simulink model "TCR_Model"  (R2026a)
settings: Solver=ode23t  StopTime=0.1  MaxStep=1e-5  RelTol=1e-4
model workspace (MAT data in the model file):
  Lr = 0.1
  PW = 60
  Rr = 0.1
  Vg = 10
  Vrms = 230
  alpha = 120
  f = 50
libraries: nesl_utility x7, fl_lib x6, ee_lib x4

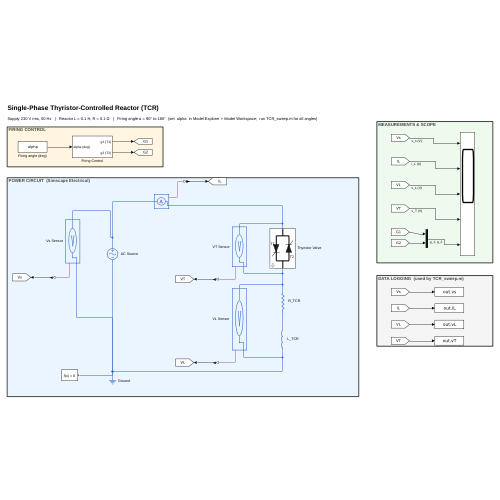
[thumbnail: Simulink's stored preview of the top-level diagram]
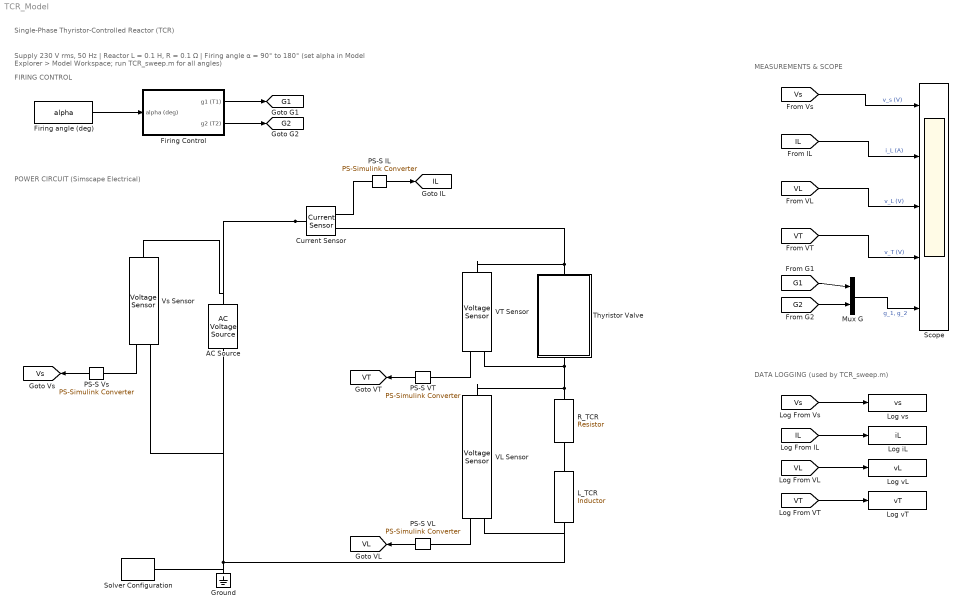
== system TCR_Model ==
  note: Single-Phase Thyristor-Controlled Reactor (TCR)
  note: Supply 230 V rms, 50 Hz | Reactor L = 0.1 H, R = 0.1 Ω | Firing angle α = 90° to 180° (set alpha in Model Explorer > Model Workspace; run TCR_sweep.m for all angles)
  note: FIRING CONTROL
  note: POWER CIRCUIT (Simscape Electrical)
  note: MEASUREMENTS & SCOPE
  note: DATA LOGGING (used by TCR_sweep.m)
  AC Source : fl_lib/Electrical/Electrical Sources/AC Voltage Source  amp=Vrms*sqrt(2) V  shift=0 deg  frequency=f Hz
  Current Sensor : fl_lib/Electrical/Electrical Sensors/Current Sensor
  Firing Control : Subsystem
  Firing angle (deg) : Constant  Value=alpha
  Ground : fl_lib/Electrical/Electrical Elements/Electrical Reference
  L_TCR : ee_lib/Passive/Inductor  l=Lr H  enable_L_tol=ee.enum.toleranceApplication.none  L_tol=20  tol_distribution=ee.enum.toleranceDistribution.uniform  nSigma=4  r=0 Ohm  g=1e-9 1/Ohm  enable_operating_limits=ee.enum.enable.no  operating_limit_action=ee.enum.passive.reportOpLim.warn  max_working_current=1 A  power_rating=1 W  i_L_specify=off  i_L_priority=High  i_L=0 A  i_L_nominal_specify=off  i_L_nominal_value=1  i_L_nominal_unit=A
  Log iL : ToWorkspace  VariableName=iL  SaveFormat=Timeseries  SampleTime=-1
  Log vL : ToWorkspace  VariableName=vL  SaveFormat=Timeseries  SampleTime=-1
  Log vT : ToWorkspace  VariableName=vT  SaveFormat=Timeseries  SampleTime=-1
  Log vs : ToWorkspace  VariableName=vs  SaveFormat=Timeseries  SampleTime=-1
  Mux G : Mux  Inputs=2
  PS-S IL : nesl_utility/PS-Simulink Converter  PhysicalDomain=network_engine_domain  SubClassName=ps_output  LeftPortType=input  RightPortType=output  PseudoPeriodic=off  Frequencies=[]  VectorFormat=inherit  Unit=inherit  AffineConversion=off
  PS-S VL : nesl_utility/PS-Simulink Converter  PhysicalDomain=network_engine_domain  SubClassName=ps_output  LeftPortType=input  RightPortType=output  PseudoPeriodic=off  Frequencies=[]  VectorFormat=inherit  Unit=inherit  AffineConversion=off
  PS-S VT : nesl_utility/PS-Simulink Converter  PhysicalDomain=network_engine_domain  SubClassName=ps_output  LeftPortType=input  RightPortType=output  PseudoPeriodic=off  Frequencies=[]  VectorFormat=inherit  Unit=inherit  AffineConversion=off
  PS-S Vs : nesl_utility/PS-Simulink Converter  PhysicalDomain=network_engine_domain  SubClassName=ps_output  LeftPortType=input  RightPortType=output  PseudoPeriodic=off  Frequencies=[]  VectorFormat=inherit  Unit=inherit  AffineConversion=off
  R_TCR : ee_lib/Passive/Resistor  R=Rr Ohm  enable_R_tol=ee.enum.toleranceApplication.none  R_tol=5  tol_distribution=ee.enum.toleranceDistribution.uniform  nSigma=4  enable_operating_limits=ee.enum.enable.no  operating_limit_action=ee.enum.passive.reportOpLim.warn  power_rating=1 W  max_working_voltage=100 V  noise_mode=ee.enum.sources.noise.Disabled  Tdevice=25 degC  sample_time=1e-3 s  repeatability=ee.enum.ic.repeatability.notRepeatable  user_seed=0  auto_seed=3002511661  power_derating_T1=70 degC  power_derating_T2=155 degC  operating_temperature_range_vec=[-50, 150] degC  alpha=3.93e-3 1/K  Tmeas=25 degC  thermal_mass=100 J/K  temperature_specify=off  temperature_priority=High  temperature=298.15 K  temperature_nominal_specify=off  temperature_nominal_value=1  temperature_nominal_unit=K
  Scope : Scope  NumInputPorts=5
      settings: ActiveDisplayString=5  Title=Gate pulses g_1, g_2  ActiveDisplayYMinimum=-1  ActiveDisplayYMaximum=11  YLabel=g
  Solver Configuration : nesl_utility/Solver Configuration  PhysicalDomain=network_engine_domain  SubClassName=solver  LeftPortType=input  RightPortType=generic  Tones=[]  Harmonics=[]  SimulateNoise=off  Profile=off  UseLocalSampling=off  EnableSwitchedLinearOptims=on  FrequencyDomain=off  UseCCode=off  RelTol=0.001  AbsTol=0.001  MinStep=1e-09  ToWorkspace=off  RevertToSquareIcSolve=off  NumHomotopyIterations=100  PhasorMode=off  PhasorModeNumHarmonics=1  ConsistencySolver=NEWTON_XTOL_AFTER_FTOL  CanonicalOrdering=CANONICAL  OptimizeIntermediates=OPTIMIZED  IndexReductionMethod=DerivativeReplacement  DoDC=off  ResidualTolerance=1e-09  ConsistencyTolSource=GLOBAL  ConsistencyAbsTol=0.001  ConsistencyRelTol=0.001  ConsistencyTolFactor=0.001  UseLocalSolver=off  LocalSolverChoice=NE_BACKWARD_EULER_ADVANCER  ResolveIndetEquations=on  FunctionEvalNumThread=1  LocalSolverSampleTime=0.001  DoFixedCost=off  MaxNonlinIter=3  MaxModeIter=2  ComputeImpulses=off  ImpulseIterations=2  LinearAlgebra=auto  LinearAlgebraNumThread=0  EquationFormulation=NE_TIME_EF  DelaysMemoryBudget=1024  AutomaticFiltering=on  FilteringTimeConstant=0.001  PartitionStorageMethod=AS_NEEDED  PartitionMemoryBudget=1024  PartitionMethod=ROBUST  MultibodyUseLocalSolver=off  MultibodyLocalSolverChoice=ODE1  MultibodyLocalSolverSampleTime=0.001
  Thyristor Valve : Subsystem
      mask help: Anti-parallel thyristor pair. Gate pulses come from Goto tags G1 and G2 (Firing Control).
      mask Display: plot([0.5 0.5],[0.82 1]); plot([0.5 0.5],[0 0.18]); plot([0.25 0.75],[0.82 0.82]); plot([0.25 0.75],[0.18 0.18]); plot([0.25 0.25],[0.18 0.82]); plot([0.75 0.75],[0.18 0.82]); patch([0.13 0.37 0.25],[0.6 0.6 0.4],[0.1 0.1 0.1]); plot([0.13 0.37],[0.4 0.4]); plot([0.25 0.08],[0.43 0.3]); patch([0.63 0.87 0.75],[0.4 0.4 0.6],[0.1 0.1 0.1]); plot([0.63 0.87],[0.6 0.6]); plot([0.75 0.92],[0.57 0.7]); text(0.03,0.62,'T1'); text(0.8,0.3,'T2');
  VL Sensor : fl_lib/Electrical/Electrical Sensors/Voltage Sensor
  VT Sensor : fl_lib/Electrical/Electrical Sensors/Voltage Sensor
  Vs Sensor : fl_lib/Electrical/Electrical Sensors/Voltage Sensor
  tag scope: G1=global, G2=global, IL=global, VL=global, VT=global, Vs=global
  wires:
  Firing angle (deg)/1 -> Firing Control/1(alpha (deg))
  Firing Control/1(g1 (T1)) -> [G1]
  Firing Control/2(g2 (T2)) -> [G2]
  PS-S IL/1 -> [IL]
  PS-S Vs/1 -> [Vs]
  PS-S VT/1 -> [VT]
  PS-S VL/1 -> [VL]
  [Vs] -> Scope/1  "v_s (V)"
  [IL] -> Scope/2  "i_L (A)"
  [VL] -> Scope/3  "v_L (V)"
  [VT] -> Scope/4  "v_T (V)"
  [G1] -> Mux G/1
  [G2] -> Mux G/2
  Mux G/1 -> Scope/5  "g_1, g_2"
  [Vs] -> Log vs/1
  [IL] -> Log iL/1
  [VL] -> Log vL/1
  [VT] -> Log vT/1
  connections:
  Current Sensor/LConn1 -- AC Source/LConn1 -- Vs Sensor/LConn1
  Thyristor Valve/LConn1 -- Current Sensor/RConn2 -- VT Sensor/LConn1
  Thyristor Valve/RConn1 -- VT Sensor/RConn2 -- R_TCR/LConn1 -- VL Sensor/LConn1
  R_TCR/RConn1 -- L_TCR/LConn1
  AC Source/RConn1 -- L_TCR/RConn1 -- VL Sensor/RConn2 -- Solver Configuration/RConn1 -- Ground/LConn1 -- Vs Sensor/RConn2
  Current Sensor/RConn1 -- PS-S IL/LConn1
  Vs Sensor/RConn1 -- PS-S Vs/LConn1
  VT Sensor/RConn1 -- PS-S VT/LConn1
  VL Sensor/RConn1 -- PS-S VL/LConn1

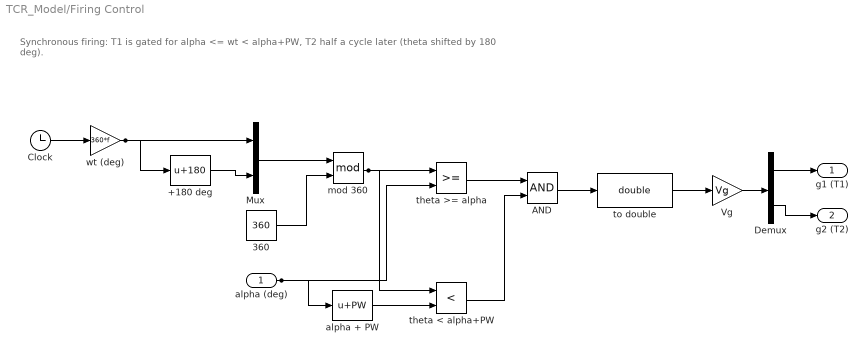
== system TCR_Model/Firing Control ==
  note: Synchronous firing: T1 is gated for alpha <= wt < alpha+PW, T2 half a cycle later (theta shifted by 180 deg).
  alpha (deg) : Inport
  +180 deg : Bias  Bias=180  SaturateOnIntegerOverflow=off
  360 : Constant  Value=360
  AND : Logic  AllPortsSameDT=off  OutDataTypeStr=boolean
  Clock : Clock
  Demux : Demux  Outputs=2
  Mux : Mux  Inputs=2
  Vg : Gain  Gain=Vg
  alpha + PW : Bias  Bias=PW  SaturateOnIntegerOverflow=off
  mod 360 : Math  Operator=mod
  theta < alpha+PW : RelationalOperator  Operator=<  OutDataTypeStr=boolean  RndMeth=Simplest  InputSameDT=off
  theta >= alpha : RelationalOperator  OutDataTypeStr=boolean  RndMeth=Simplest  InputSameDT=off
  to double : DataTypeConversion  OutDataTypeStr=double  SaturateOnIntegerOverflow=off  RndMeth=Floor
  wt (deg) : Gain  Gain=360*f
  g1 (T1) : Outport
  g2 (T2) : Outport  Port=2
  wires:
  Demux/2 -> g2 (T2)/1
  Demux/1 -> g1 (T1)/1
  Clock/1 -> wt (deg)/1
  +180 deg/1 -> Mux/2
  wt (deg)/1 -> +180 deg/1, Mux/1
  mod 360/1 -> theta < alpha+PW/1, theta >= alpha/1
  to double/1 -> Vg/1
  alpha + PW/1 -> theta < alpha+PW/2
  alpha (deg)/1 -> alpha + PW/1, theta >= alpha/2
  360/1 -> mod 360/2
  theta >= alpha/1 -> AND/1
  theta < alpha+PW/1 -> AND/2
  Mux/1 -> mod 360/1
  AND/1 -> to double/1
  Vg/1 -> Demux/1

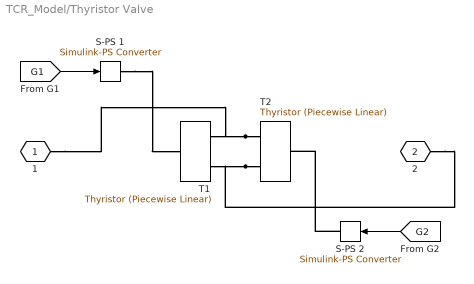
== system TCR_Model/Thyristor Valve ==
  S-PS 1 : nesl_utility/Simulink-PS Converter  PhysicalDomain=network_engine_domain  SubClassName=ps_input  LeftPortType=input  RightPortType=output  PseudoPeriodic=off  Frequencies=[]  NoiseDistribution=none  NoiseParameters=[]  Unit=1  AffineConversion=off  FilteringAndDerivatives=provide  SimscapeFilterOrder=1  InputFilterTimeConstant=0.001  UdotUserProvided=0
  S-PS 2 : nesl_utility/Simulink-PS Converter  PhysicalDomain=network_engine_domain  SubClassName=ps_input  LeftPortType=input  RightPortType=output  PseudoPeriodic=off  Frequencies=[]  NoiseDistribution=none  NoiseParameters=[]  Unit=1  AffineConversion=off  FilteringAndDerivatives=provide  SimscapeFilterOrder=1  InputFilterTimeConstant=0.001  UdotUserProvided=0
  T1 : ee_lib/Semiconductors & Converters/Thyristor (Piecewise Linear)  port_option=ee.enum.controlport.ps  Vf=0.8 V  Ron=0.001 Ohm  Goff=1e-5 1/Ohm  Vgt=6 V  Ih=1e-3 A  diode_param=ee.enum.semiconductors.protectionDiode.external  diode_Vf=0.8 V  diode_Ron=0.001 Ohm  diode_Goff=1e-5 1/Ohm  diode_C=50e-9 F  diode_iRM=-235 A  diode_iF=300 A  diode_idot=-50 A/us  diode_trr_param=ee.enum.converters.diodetrr.trr_factor  diode_trr_factor=3  diode_trr=15 us  diode_Qrr=1500 s*uA  iak_specify=off  iak_priority=None  iak=0 A  iak_nominal_specify=off  iak_nominal_value=1  iak_nominal_unit=A  vak_specify=off  vak_priority=None  vak=0 V  vak_nominal_specify=off  vak_nominal_value=1  vak_nominal_unit=V  vgk_specify=off  vgk_priority=None  vgk=0 V  vgk_nominal_specify=off  vgk_nominal_value=1  vgk_nominal_unit=V  thermal_loss_option=ee.enum.converters.thermalLossOption.constantvalues  Von_data=[0, .1, .6, .8, 1, 1.3, 1.6, 2, 2.4; 0, .1, .7, 1, 1.2, 1.5, 1.9, 2.4, 2.8] V  Tj=[298.15, 398.15] K  Iout_data=[0, .1, 1, 5, 10, 20, 40, 70, 100] A  Eon_data=[0, .0024, .024, .12, .2, .48, 1.04, 2.16, 3.24; 0, .003, .03, .15, .25, .6, 1.3, 2.7, 4.05] * 1e-3 J  Tj_loss=[298.15, 398.15] K  Iout_data_loss=[0, .1, 1, 5, 10, 20, 40, 70, 100] A  Eon_scalar=22.86e-3 J  Eoff_natural_commutation=10e-3 J  Voff=300 V  Iout_scalar=600 A  onCurrentMeasDelay=1e-4 s  diodeModelType=ee.enum.converters.diodeModelType.pwl  diodeTableType=ee.enum.diode.tableType.IfMat  diode_IfMat=[.07, .12, .19, 1.75, 4.24, 7.32, 11.2; .16, .3, .72, 2.14, 4.02, 6.35, 9.12] A  diode_VfMat=[.9, 1.15, 1.25, 1.5, 1.75, 2.17, 2.6, 2.85; .58, .68, .75, 1.1, 1.38, 1.77, 2.27, 2.7] V  diode_TjVec=[25, 125] degC  diode_VfVec=[.5, .7, .9, 1.3, 1.7, 2.1, 2.5] V  diode_IfVec=[.1, .2, .5, 1, 2, 4, 7, 10] A  diode_rec_loss_model=ee.enum.diode.reverseRecoveryModel.fixed  diode_ErecVal=0 J  diode_scaleWithIandV=true  diode_ErecMat=zeros(2, 3) J  diode_TjrecVec=[298.15, 398.15] K  diode_IfrecVec=[.1, 1, 10] A  diode_IrecVal=10 A  diode_VrecVal=10 V  diode_tFilter=1 / 1000 / 100 s  thermal_network_parameterization=ee.enum.thermalNetworkTopology.external  Rth=[.08, .5] K/W  Rth_Cauer=[.08, .1, .5] K/W  Rth_Foster=[.08, .14, .22, .16] K/W  thermal_mass_parameterization=ee.enum.thermalNetwork.timeconstant  thermal_mass=[.01, .5] J/K  thermal_mass_Cauer=[.01, .1, .5] J/K  thermal_mass_Foster=[.001, .005, .05, .5] J/K  thermal_time_constant=[.001, .2] s  thermal_time_constant_Cauer=[.001, .1, .2] s  thermal_time_constant_Foster=[7e-05, .0007, .01, .08] s  thermal_mass_initial_temperatures=[25, 25] degC  thermal_mass_initial_temperatures_Cauer=[25, 25, 25] degC  junction_thermal_mass=0.01 J/K  Tvec_initial_Foster=[25, 25, 25, 25] degC  junction_temperature_specify=off  junction_temperature_priority=None  junction_temperature=25 degC  junction_temperature_nominal_specify=off  junction_temperature_nominal_value=1  junction_temperature_nominal_unit=degC  Qj_specify=off  Qj_priority=None  Qj=0 W  Qj_nominal_specify=off  Qj_nominal_value=1  Qj_nominal_unit=W  accumulatedSwitchingLosses_specify=off  accumulatedSwitchingLosses_priority=None  accumulatedSwitchingLosses=0 J
  T2 : ee_lib/Semiconductors & Converters/Thyristor (Piecewise Linear)  port_option=ee.enum.controlport.ps  Vf=0.8 V  Ron=0.001 Ohm  Goff=1e-5 1/Ohm  Vgt=6 V  Ih=1e-3 A  diode_param=ee.enum.semiconductors.protectionDiode.external  diode_Vf=0.8 V  diode_Ron=0.001 Ohm  diode_Goff=1e-5 1/Ohm  diode_C=50e-9 F  diode_iRM=-235 A  diode_iF=300 A  diode_idot=-50 A/us  diode_trr_param=ee.enum.converters.diodetrr.trr_factor  diode_trr_factor=3  diode_trr=15 us  diode_Qrr=1500 s*uA  iak_specify=off  iak_priority=None  iak=0 A  iak_nominal_specify=off  iak_nominal_value=1  iak_nominal_unit=A  vak_specify=off  vak_priority=None  vak=0 V  vak_nominal_specify=off  vak_nominal_value=1  vak_nominal_unit=V  vgk_specify=off  vgk_priority=None  vgk=0 V  vgk_nominal_specify=off  vgk_nominal_value=1  vgk_nominal_unit=V  thermal_loss_option=ee.enum.converters.thermalLossOption.constantvalues  Von_data=[0, .1, .6, .8, 1, 1.3, 1.6, 2, 2.4; 0, .1, .7, 1, 1.2, 1.5, 1.9, 2.4, 2.8] V  Tj=[298.15, 398.15] K  Iout_data=[0, .1, 1, 5, 10, 20, 40, 70, 100] A  Eon_data=[0, .0024, .024, .12, .2, .48, 1.04, 2.16, 3.24; 0, .003, .03, .15, .25, .6, 1.3, 2.7, 4.05] * 1e-3 J  Tj_loss=[298.15, 398.15] K  Iout_data_loss=[0, .1, 1, 5, 10, 20, 40, 70, 100] A  Eon_scalar=22.86e-3 J  Eoff_natural_commutation=10e-3 J  Voff=300 V  Iout_scalar=600 A  onCurrentMeasDelay=1e-4 s  diodeModelType=ee.enum.converters.diodeModelType.pwl  diodeTableType=ee.enum.diode.tableType.IfMat  diode_IfMat=[.07, .12, .19, 1.75, 4.24, 7.32, 11.2; .16, .3, .72, 2.14, 4.02, 6.35, 9.12] A  diode_VfMat=[.9, 1.15, 1.25, 1.5, 1.75, 2.17, 2.6, 2.85; .58, .68, .75, 1.1, 1.38, 1.77, 2.27, 2.7] V  diode_TjVec=[25, 125] degC  diode_VfVec=[.5, .7, .9, 1.3, 1.7, 2.1, 2.5] V  diode_IfVec=[.1, .2, .5, 1, 2, 4, 7, 10] A  diode_rec_loss_model=ee.enum.diode.reverseRecoveryModel.fixed  diode_ErecVal=0 J  diode_scaleWithIandV=true  diode_ErecMat=zeros(2, 3) J  diode_TjrecVec=[298.15, 398.15] K  diode_IfrecVec=[.1, 1, 10] A  diode_IrecVal=10 A  diode_VrecVal=10 V  diode_tFilter=1 / 1000 / 100 s  thermal_network_parameterization=ee.enum.thermalNetworkTopology.external  Rth=[.08, .5] K/W  Rth_Cauer=[.08, .1, .5] K/W  Rth_Foster=[.08, .14, .22, .16] K/W  thermal_mass_parameterization=ee.enum.thermalNetwork.timeconstant  thermal_mass=[.01, .5] J/K  thermal_mass_Cauer=[.01, .1, .5] J/K  thermal_mass_Foster=[.001, .005, .05, .5] J/K  thermal_time_constant=[.001, .2] s  thermal_time_constant_Cauer=[.001, .1, .2] s  thermal_time_constant_Foster=[7e-05, .0007, .01, .08] s  thermal_mass_initial_temperatures=[25, 25] degC  thermal_mass_initial_temperatures_Cauer=[25, 25, 25] degC  junction_thermal_mass=0.01 J/K  Tvec_initial_Foster=[25, 25, 25, 25] degC  junction_temperature_specify=off  junction_temperature_priority=None  junction_temperature=25 degC  junction_temperature_nominal_specify=off  junction_temperature_nominal_value=1  junction_temperature_nominal_unit=degC  Qj_specify=off  Qj_priority=None  Qj=0 W  Qj_nominal_specify=off  Qj_nominal_value=1  Qj_nominal_unit=W  accumulatedSwitchingLosses_specify=off  accumulatedSwitchingLosses_priority=None  accumulatedSwitchingLosses=0 J
  1 : PMIOPort  Side=Left
  2 : PMIOPort  Port=2  Side=Right
  wires:
  [G1] -> S-PS 1/1
  [G2] -> S-PS 2/1
  connections:
  S-PS 1/RConn1 -- T1/LConn1
  S-PS 2/RConn1 -- T2/LConn1
  T2/RConn2 -- T1/RConn1 -- 1/RConn1
  T2/RConn1 -- T1/RConn2 -- 2/RConn1
